simulink model "KT_Robot_Robustness"  (R2025b)
settings: Solver=FixedStepDiscrete  StartTime=0.0  StopTime=tEnd  FixedStep=Ts  RelTol=1e-3
model workspace (MAT data in the model file):
  Ts = 0.05
  impact = [0; 0.1; 0.174532925199; 4; 1; 0.4; 0.04; -0.04; 2; 3.5]
  initialPose = [0; -0.6; 0]
  noise = [-0.649013765191 1.18116604197 -0.758453297284 -1.1096130385 -0.845551240008 -0.572664866458 -0.558680764474 0.17838022585 -0.196861446476 0.586442621667 -0.851886969622 0.800320709802 ... (7323 elements, 3x2441)]
  pathData = [0 4 4 8 8 0 0 3 3 6 0 4 ... (20 elements, 5x4)]
  robot = [0.05; 0.3; 12; 2]
  settings = [0.55; 0.5; 0.05; 1; 1.308996939; 2; 0; 0.12; 0.05; 2400]
  tEnd = 122
(part 2 of 2)

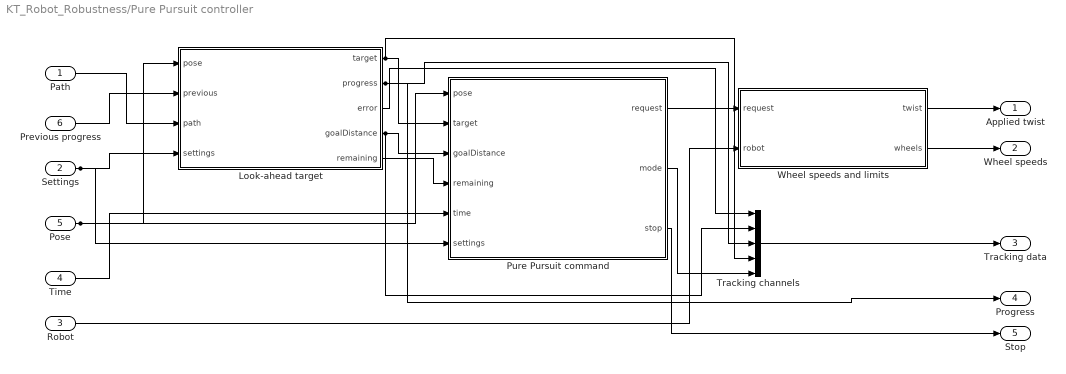
== system KT_Robot_Robustness/Pure Pursuit controller ==
  Path : Inport
  Settings : Inport  Port=2
  Robot : Inport  Port=3
  Time : Inport  Port=4
  Pose : Inport  Port=5
  Previous progress : Inport  Port=6
  Look-ahead target : MATLAB Function  TreatAsAtomicUnit=on
  Pure Pursuit command : MATLAB Function  TreatAsAtomicUnit=on
  Tracking channels : Mux  Inputs=[1 1 1 2 1]
  Wheel speeds and limits : MATLAB Function  TreatAsAtomicUnit=on
  Applied twist : Outport
  Wheel speeds : Outport  Port=2
  Tracking data : Outport  Port=3
  Progress : Outport  Port=4
  Stop : Outport  Port=5
  wires:
  Pure Pursuit command/3(stop) -> Stop/1
  Tracking channels/1 -> Tracking data/1
  Pure Pursuit command/2(mode) -> Tracking channels/5
  Look-ahead target/2(progress) -> Progress/1, Tracking channels/3
  Look-ahead target/3(error) -> Tracking channels/1
  Wheel speeds and limits/2(wheels) -> Wheel speeds/1
  Wheel speeds and limits/1(twist) -> Applied twist/1
  Robot/1 -> Wheel speeds and limits/2(robot)
  Pure Pursuit command/1(request) -> Wheel speeds and limits/1(request)
  Time/1 -> Pure Pursuit command/5(time)
  Look-ahead target/5(remaining) -> Pure Pursuit command/4(remaining)
  Look-ahead target/4(goalDistance) -> Tracking channels/2, Pure Pursuit command/3(goalDistance)
  Look-ahead target/1(target) -> Tracking channels/4, Pure Pursuit command/2(target)
  Settings/1 -> Pure Pursuit command/6(settings), Look-ahead target/4(settings)
  Path/1 -> Look-ahead target/3(path)
  Previous progress/1 -> Look-ahead target/2(previous)
  Pose/1 -> Pure Pursuit command/1(pose), Look-ahead target/1(pose)

== matlab function KT_Robot_Robustness/Settling check ==
  data: terminal input size=2; stop output; wheels input size=2; event input size=3; time input; dt input
function stop = kt_robust_stop(terminal,wheels,event,time,dt)
% End when settled, or after two seconds even if the plant is still moving.
settled = max(abs(wheels)) <= .1 && event(3) == 0;
tailExpired = round((time-terminal(2))/dt)>=round(2/dt);
stop = terminal(2)>=0 && (settled || tailExpired);
end

== matlab function KT_Robot_Robustness/Pure Pursuit controller/Look-ahead target ==
  data: pose input; target output; previous input; path input; settings input; progress output; error output; goalDistance output; remaining output
function [target, progress, error, goalDistance, remaining] = pp_target(pose, previous, path, settings)
% Find the first forward circle intersection on the reference polyline.
xy = pose(1:2);
n = size(path,1);
total = path(n,3);
lookahead = settings(1);
progress = project(xy, path, previous, min(total, previous + max(2*lookahead,1)));
[~, error] = project(xy, path, 0, total);
goal = path(n,1:2).';
goalDistance = norm(goal - xy);
remaining = total - progress;
target = goal;
if remaining <= lookahead
    return
end

for i = 1:n-1
    if path(i+1,3) <= progress
        continue
    end
    p = path(i,1:2).';
    d = path(i+1,1:2).' - p;
    length = path(i,4);
    q = p - xy;
    a = dot(d,d);
    b = 2*dot(q,d);
    c = dot(q,q) - lookahead^2;
    disc = b*b - 4*a*c;
    if disc < 0
        continue
    end
    root = sqrt(disc);
    for u = [(-b-root)/(2*a), (-b+root)/(2*a)]
        if u >= 0 && u <= 1 && path(i,3) + u*length > progress + 1e-8
            target = p + u*d;
            return
        end
    end
end

s = min(progress + lookahead,total);
for i = 1:n-1
    if s < path(i+1,3) || i == n-1
        p = path(i,1:2).';
        d = path(i+1,1:2).' - p;
        target = p + ((s-path(i,3))/path(i,4))*d;
        return
    end
end
end

function [s, distance] = project(xy, path, first, last)
% Strict improvement preserves the first segment in a projection tie.
s = first;
distance = inf;
for i = 1:size(path,1)-1
    if path(i+1,3) < first || path(i,3) > last
        continue
    end
    p = path(i,1:2).';
    d = path(i+1,1:2).' - p;
    length = path(i,4);
    u = dot(xy-p,d)/length^2;
    low = max(0,(first-path(i,3))/length);
    high = min(1,(last-path(i,3))/length);
    u = min(max(u,low),high);
    e = norm(p + u*d - xy);
    if e < distance
        distance = e;
        s = path(i,3) + u*length;
    end
end
end

== matlab function KT_Robot_Robustness/Localization ==
  data: pose input size=3; measured output size=3; event input size=3; time input; dt input; impact input; noise input
function measured = kt_robust_sensor(pose,event,time,dt,impact,noise)
% Add Gaussian noise, delay by whole samples, and hold during outages.
persistent history lastValid
if isempty(history)
    history = zeros(3,4);
    lastValid = zeros(3,1);
end
if round(time/dt) == 0
    history(:,:) = repmat(pose,1,4);
    lastValid = pose;
end
sample = pose + impact(1:3).*noise(:,min(round(time/dt)+1,size(noise,2)));
delay = impact(4);
delivered = sample;
if delay > 0
    delivered = history(:,delay);
end
history = [sample history(:,1:3)];
if event(2) == 0
    lastValid = delivered;
end
measured = lastValid;
end

== matlab function KT_Robot_Robustness/Pure Pursuit controller/Pure Pursuit command ==
  data: pose input; request output; target input; goalDistance input; remaining input; time input; settings input; mode output; stop output
function [request, mode, stop] = pp_command(pose, target, goalDistance, remaining, time, settings)
% Modes: pursuit (0), alignment (1), goal (2), and timeout (3).
lookahead = settings(1);
nearEnd = remaining <= lookahead;
reached = nearEnd && goalDistance <= settings(3);
timeout = round(time/settings(9)) >= settings(10);
stop = reached || timeout;
request = zeros(2,1);
if stop
    mode = 3;
    if reached
        mode = 2;
    end
    return
end

offset = target - pose(1:2);
theta = pose(3);
alpha = mod(atan2(offset(2),offset(1)) - theta + pi,2*pi) - pi;
if abs(alpha) > settings(5)
    mode = 1;
    request(2) = settings(6)*alpha;
    return
end

mode = 0;
v = settings(2);
if nearEnd
    v = min(v,settings(4)*goalDistance);
end
yBody = -sin(theta)*offset(1) + cos(theta)*offset(2);
kappa = 2*yBody/max(dot(offset,offset),1e-12);
if settings(7) == 1
    v = min(v,sqrt(settings(8)/max(abs(kappa),1e-12)));
end
request = [v; v*kappa];
end

== matlab function KT_Robot_Robustness/Pure Pursuit controller/Wheel speeds and limits ==
  data: request input; twist output; robot input; wheels output
function [twist,wheels] = pp_wheels(request, robot)
% Limit yaw first, then both wheels together to retain curvature.
radius = robot(1);
track = robot(2);
limited = request/max(1,abs(request(2))/robot(4));
v = limited(1);
omega = limited(2);
left = (v-track*omega/2)/radius;
right = (v+track*omega/2)/radius;
wheels = [left;right]/max([1,abs(left)/robot(3),abs(right)/robot(3)]);
twist = [radius*(wheels(1)+wheels(2))/2; radius*(wheels(2)-wheels(1))/track];
end

== matlab function KT_Robot_Robustness/Goal decision latch ==
  data: wheels input size=2; command output size=2; tracking input size=6; time input; terminal output size=2
function [command,terminal] = kt_robust_command(wheels,tracking,time)
% Latch the first terminal controller decision and hold zero thereafter.
persistent decision decidedAt
if isempty(decision)
    decision = 0;
    decidedAt = -1;
end
mode = tracking(6);
if decision == 0 && mode >= 2
    decision = mode;
    decidedAt = time;
end
command = [wheels(1); wheels(2)];
if decision ~= 0
    command = zeros(2,1);
    mode = decision;
end
terminal = [mode;decidedAt];
end

== matlab function KT_Robot_Robustness/Motor and slip model ==
  data: command input size=2; realWheels output size=2; robot input size=4; impact input size=10; event input size=3; time input; dt input; body output size=3; slip output size=2
function [realWheels,body,slip] = kt_robust_actuator(command,robot,impact,event,time,dt)
% First-order wheel response plus radius mismatch and local translational slip.
persistent previous
if isempty(previous)
    previous = zeros(2,1);
end
realWheels = command;
if impact(6) > 0
    decay = exp(-dt/impact(6));
    realWheels = decay*previous + (1-decay)*command;
end
previous = realWheels;
rim = robot(1)*(1+impact(7:8)).*realWheels;
slip = zeros(2,1);
if event(3) ~= 0
    elapsed = round((time-event(1))/dt)*dt;
    slip = impact(9)*[.03*sin(1.2*elapsed+.045408*pi); ...
                      .05*cos(1.2*elapsed-.00459*pi)];
end
body = [(rim(1)+rim(2))/2 + slip(1); slip(2); (rim(2)-rim(1))/robot(2)];
end

== matlab function KT_Robot_Robustness/Integrate true pose ==
  data: pose input size=3; nextPose output size=3; body input size=3; dt input
function nextPose = kt_robust_motion(pose,body,dt)
% Integrate constant body-frame longitudinal and lateral speeds for a sample.
theta = pose(3);
v = body(1);
vy = body(2);
omega = body(3);
nextTheta = theta + omega*dt;
if abs(omega) < 1e-10
    displacement = v*[cos(theta);sin(theta)]*dt ...
        + vy*[-sin(theta);cos(theta)]*dt;
else
    ds = sin(nextTheta)-sin(theta);
    dc = cos(theta)-cos(nextTheta);
    displacement = (v/omega)*[ds;dc] + (vy/omega)*[-dc;ds];
end
nextPose = [pose(1:2) + displacement; mod(nextTheta+pi,2*pi)-pi];
end

== matlab function KT_Robot_Robustness/True path geometry ==
  data: pose input size=3; geometry output size=3; path input; time input; impact input; dt input; event output size=3
function [geometry,event] = kt_robust_truth(pose,path,time,impact,dt)
% Ground-truth path geometry and the first threshold crossing.
persistent eventStep
if isempty(eventStep)
    eventStep = -1;
end
xy = pose(1:2);
progress = 0;
error = inf;
for i = 1:size(path,1)-1
    p = path(i,1:2).';
    d = path(i+1,1:2).' - p;
    length = path(i,4);
    fraction = min(max(dot(xy-p,d)/length^2,0),1);
    gap = norm(p+fraction*d-xy);
    if gap < error
        progress = path(i,3) + fraction*length;
        error = gap;
    end
end
goalDistance = norm(path(end,1:2).' - xy);
step = round(time/dt);
if eventStep < 0 && progress > impact(10)
    eventStep = step;
end
event = [-1;0;0];
if eventStep >= 0
    elapsed = (step-eventStep)*dt;
    event = [eventStep*dt; double(elapsed < impact(5)); ...
        double(impact(9) ~= 0 && elapsed < 3)];
end
geometry = [progress;error;goalDistance];
end
